simulink model "SCBuckHybridBuck_COMPEL23"  (R2022b)
settings: Solver=VariableStepAuto  StartTime=0.0  StopTime=10.0  RelTol=1e-3
StopFcn:
  | ton = .075e-6;
  | toff = .175e-6;
  | dtBuck = .01e-6;
  | dtSC = .001e-6;
  | 
  | p = [1/2 0 1/2];
  | d = [0 dtSC 0];
  | ts = [ton*p+d dtBuck toff*p+d dtBuck ton*p+d dtBuck toff*p+d dtBuck ton*p+d dtBuck toff*p+d dtBuck];
  | doff =        [ 0 0 0    1       1 1];
  |               %3 4 5    6      10 11
  | DCbuckswvec = [repmat([1 0 0    1       1 0],3,1);
  |                0 0 0    1       1 0;
  |                repmat(doff,3,1);
  |                0 0 0    1       0 1;
  |                repmat([0 1 0    1       0 1],3,1);
  |                0 0 0    1       0 1;
  |                repmat(doff,3,1);
  |                0 0 0    0       1 1;
  |                repmat([0 0 1    0       1 1],3,1);
  |                0 0 0    0       1 1;
  |                repmat(doff,3,1)
  |                0 0 0    1       1 0];
  | 
  | SCBucksswvec = [repmat([1 0 0],11+8,1);
  |                 0 0 0;
  |                 repmat([0 1 1],3,1);
  |                 0 0 0];
  | 
  | SCBucksswvec = circshift(SCBucksswvec,1);
  | 
  | swvec = [];
  | 
  | swvec(:,1:4) = DCbuckswvec(:,1:4);
  | swvec(:,8:9) = DCbuckswvec(:,5:6);
  | swvec(:,5:7) = circshift(SCBucksswvec(:,1:3),1);
  | swvec(:,10:12) = circshift(SCBucksswvec(:,1:3),9);
  | swvec(:,13:15) = circshift(SCBucksswvec(:,1:3),17);
  | 
  | % Io = Iout;
  | 
  | % Lr = 0;
  | % Lf = 0.25e-6;
  | % swvec = [0 0; 0 1 ; 0 0; 1 0];
  | % Ts = [5e-6 .2e-6 1e-6];
  | % Ts = Ts(startPoint);
  | % ts = [.05 .8 .05 .1]*Ts;
  | % origts = ts;
  | % swvec = [0 1 ;  1 0];
  | % Ts = [5e-6 .1e-6 1e-6];
  | % Ts = Ts(startPoint);
  | % ts = [ .9  .1]*Ts;
  | 
  | % data(:,1) = data(:,1)/10; %ron
  | % data(:,2) = data(:,2)/1e8; % Coss
  | 
  | swvec = [swvec, zeros(size(swvec))];
  | 
  | Nsw = 15;
  | for i = 3:Nsw+2
  |     evalin('base',['ron' num2str(i) ' = 1e-3']);
  |     evalin('base',['Coss' num2str(i) ' = 1e-9']);
  | end
  | 
  | Vf = .25;
  | us = [48 10 Vf*ones(1,Nsw)];
  | 
  | assignin('base','swvec', swvec);
  | assignin('base','us', us);
  | assignin('base','ts', ts);
undefined symbols (not defined in the file): plecs
settings Model: Creator=dcostine  LastModifiedBy=dcostine
settings DebuggingCC: UnconnectedInputMsg=warning  UnconnectedOutputMsg=warning  UnconnectedLineMsg=warning
settings ModelReferenceCC: EnableRefExpFcnMdlSchedulingChecks=on
settings RTWCC: DLArmComputeVersion=19.05

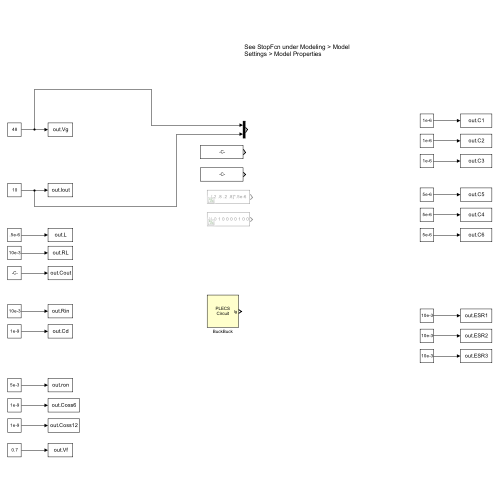
[thumbnail: Simulink's stored preview of the top-level diagram]
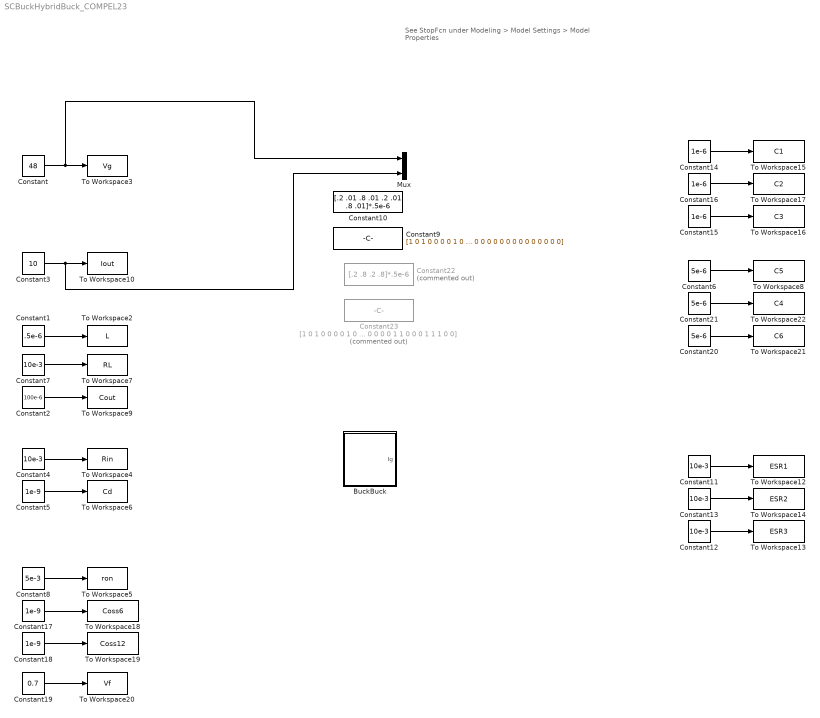
== system SCBuckHybridBuck_COMPEL23 ==
  note: See StopFcn under Modeling > Model Settings > Model Properties
  BuckBuck : Subsystem  LoadFcn=plecs('sl', 200);  InitFcn=plecs('sl', 214);  StartFcn=plecs('sl', 208);  StopFcn=plecs('sl', 209);  mask(PlecsCircuit){PLECSData=<binary blob, 5548 chars, not shown>}
      mask prompts: PLECSData "PLECS Data (Do not delete or modify!)"
      mask init:
      | % PLACE CUSTOM INITIALIZATIONS ABOVE
      | % DO NOT REMOVE
      | plecs('sl', 215);
      | % DO NOT REMOVE
      settings: CopyFcn=plecs('sl', 203);  DeleteFcn=plecs('sl', 205);  UndoDeleteFcn=plecs('sl', 206);  PreSaveFcn=plecs('sl', 211);  PostSaveFcn=plecs('sl', 201);  NameChangeFcn=plecs('sl', 210);  DestroyFcn=plecs('sl', 207);  PreCopyFcn=plecs('sl', 216);  OpenFcn=plecs('sl', 202);  ErrorFcn=plerrorfcn
      mask Help: web(['file:///' fullfile(plecsdoc, 'creatingacircuit.html')])
      mask Display: disp('PLECS\nCircuit')
  Constant : Constant  Value=48
  Constant1 : Constant  Value=.5e-6
  Constant10 : Constant  Value=[.2 .01 .8 .01 .2 .01 .8 .01]*.5e-6
  Constant{4,7,11..13} (5 alike) : Constant  Value=10e-3
  Constant14 : Constant  Value=1e-6
  Constant15 : Constant  Value=1e-6
  Constant16 : Constant  Value=1e-6
  Constant17 : Constant  Value=1e-9
  Constant18 : Constant  Value=1e-9
  Constant19 : Constant  Value=0.7
  Constant2 : Constant  Value=100e-6
  Constant20 : Constant  Value=5e-6
  Constant21 : Constant  Value=5e-6
  Constant22 : Constant  Commented=on  Value=[.2 .8 .2 .8]*.5e-6
  Constant23 : Constant  Commented=on  Value="[1 0 1 0 0 0 0 1 0 0 0 0 0 0 0; 0 0 0 1 0 0 0 1 1 0 0 0 0 0 0; 0 1 0 1 0 0 0 0 1 0 0 0 0 0 0; 0 0 0 1 0 0 0 1 1 0 0 0 0 0 0; ] + [0 0 0 0 1 0 0 0 0 1 0 0 0 1 1; 0 0 0 0 1 0 0 0 0 1 0 0 0 1 1; 0 0 0 0 0 1 1 0 0 0 1 1 1 0 0;  0 0 0 0 0 1 1 0 0 0 1 1 1 0 0]"
  Constant3 : Constant  Value=10
  Constant5 : Constant  Value=1e-9
  Constant6 : Constant  Value=5e-6
  Constant8 : Constant  Value=5e-3
  Constant9 : Constant  Value="[1 0 1 0 0 0 0 1 0 0 0 0 0 0 0; 0 0 0 0 0 0 0 0 0 0 0 0 0 0 0; 0 0 0 1 0 0 0 1 1 0 0 0 0 0 0; 0 0 0 0 0 0 0 0 0 0 0 0 0 0 0; 0 1 0 1 0 0 0 0 1 0 0 0 0 0 0; 0 0 0 0 0 0 0 0 0 0 0 0 0 0 0; 0 0 0 1 0 0 0 1 1 0 0 0 0 0 0; 0 0 0 0 0 0 0 0 0 0 0 0 0 0 0;] + [0 0 0 0 1 0 0 0 0 1 0 0 0 1 1; 0 0 0 0 1 0 0 0 0 1 0 0 0 1 1; 0 0 0 0 1 0 0 0 0 1 0 0 0 1 1;  0 0 0 0 0 0 0 0 0 0 0 0 0 0 0; 0 0 0 0 0 1 1 0 0 0 1 1 1 0 0;  0 0 0 0 0 1 1 0 0 0 1 1 1 0 0; 0 0 0 0 0 1 1 0 0 0 1 1 1 0 0; 0 0 0 0 0 0 0 0 0 0 0 0 0 0 0]"
  Mux : Mux  Inputs=2
  To Workspace10 : ToWorkspace  VariableName=Iout  SampleTime=-1
  To Workspace12 : ToWorkspace  VariableName=ESR1  SampleTime=-1
  To Workspace13 : ToWorkspace  VariableName=ESR3  SampleTime=-1
  To Workspace14 : ToWorkspace  VariableName=ESR2  SampleTime=-1
  To Workspace15 : ToWorkspace  VariableName=C1  SampleTime=-1
  To Workspace16 : ToWorkspace  VariableName=C3  SampleTime=-1
  To Workspace17 : ToWorkspace  VariableName=C2  SampleTime=-1
  To Workspace18 : ToWorkspace  VariableName=Coss6  SampleTime=-1
  To Workspace19 : ToWorkspace  VariableName=Coss12  SampleTime=-1
  To Workspace2 : ToWorkspace  VariableName=L  SampleTime=-1
  To Workspace20 : ToWorkspace  VariableName=Vf  SampleTime=-1
  To Workspace21 : ToWorkspace  VariableName=C6  SampleTime=-1
  To Workspace22 : ToWorkspace  VariableName=C4  SampleTime=-1
  To Workspace3 : ToWorkspace  VariableName=Vg  SampleTime=-1
  To Workspace4 : ToWorkspace  VariableName=Rin  SampleTime=-1
  To Workspace5 : ToWorkspace  VariableName=ron  SampleTime=-1
  To Workspace6 : ToWorkspace  VariableName=Cd  SampleTime=-1
  To Workspace7 : ToWorkspace  VariableName=RL  SampleTime=-1
  To Workspace8 : ToWorkspace  VariableName=C5  SampleTime=-1
  To Workspace9 : ToWorkspace  VariableName=Cout  SampleTime=-1
  wires:
  Constant1/1 -> To Workspace2/1
  Constant/1 -> Mux/1, To Workspace3/1
  Constant8/1 -> To Workspace5/1
  Constant2/1 -> To Workspace9/1
  Constant5/1 -> To Workspace6/1
  Constant3/1 -> Mux/2, To Workspace10/1
  Constant4/1 -> To Workspace4/1
  Constant11/1 -> To Workspace12/1
  Constant12/1 -> To Workspace13/1
  Constant13/1 -> To Workspace14/1
  Constant15/1 -> To Workspace16/1
  Constant16/1 -> To Workspace17/1
  Constant14/1 -> To Workspace15/1
  Constant17/1 -> To Workspace18/1
  Constant18/1 -> To Workspace19/1
  Constant7/1 -> To Workspace7/1
  Constant19/1 -> To Workspace20/1
  Constant6/1 -> To Workspace8/1
  Constant20/1 -> To Workspace21/1
  Constant21/1 -> To Workspace22/1

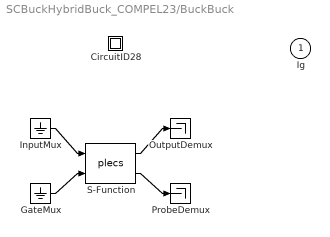
== system SCBuckHybridBuck_COMPEL23/BuckBuck ==
  " CircuitID28 " : Subsystem
  " GateMux " : Ground
  " InputMux " : Ground
  " OutputDemux " : Terminator
  " ProbeDemux " : Terminator
  " S-Function " : S-Function  FunctionName=plecs  SFunctionDeploymentMode=off  EnableBusSupport=off
  Ig : Outport  PortDimensions=1  VectorParamsAs1DForOutWhenUnconnected=off
  wires:
  " InputMux "/1 -> " S-Function "/1
  " GateMux "/1 -> " S-Function "/2
  " S-Function "/1 -> " OutputDemux "/1
  " S-Function "/2 -> " ProbeDemux "/1

== system SCBuckHybridBuck_COMPEL23/BuckBuck/ CircuitID28  ==
